simulink model "odrive_foc"  (R2024b)
settings: Solver=FixedStepDiscrete  StartTime=0  StopTime=4  FixedStep=5e-05  RelTol=1e-3
model workspace (MAT data in the model file):
  demo_load_nm = 0.0014
  demo_mode = 2
  demo_target = 2
  motor.R_ohm = 8
  motor.L_h = 0.00425
  motor.pole_pairs = 7
  motor.flux_wb = 0.003
  motor.inertia_kgm2 = 3e-05
  motor.damping_nms = 0.0003
undefined symbols (not defined in the file or in its folder): DiscIntNeverNeededParam
libraries: simulink x9
Description:
  | ODrive 3.6 three-loop bench. Export the FOC Motion Controller subsystem to the STM32.
settings Model: Creator=ODrive 3.6 Simulink FOC contributors  LastModifiedBy=ODrive 3.6 Simulink FOC contributors
settings DebuggingCC: AlgebraicLoopMsg=error

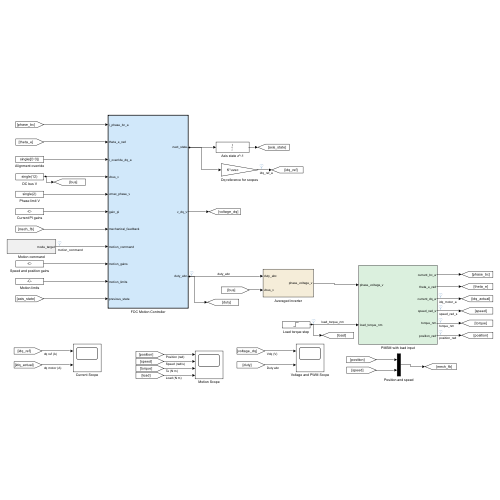
[thumbnail: Simulink's stored preview of the top-level diagram]
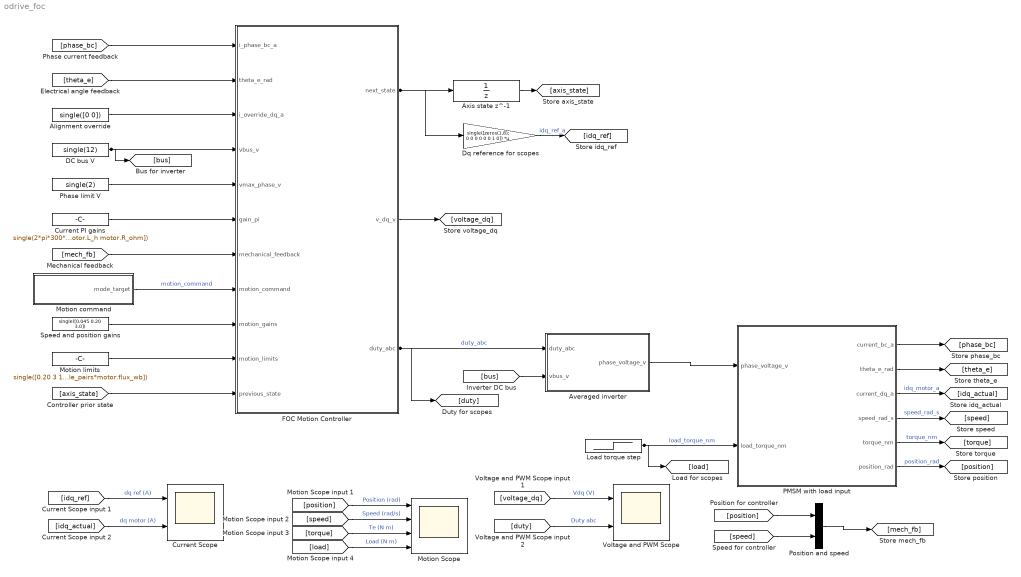
== system odrive_foc ==
  Alignment override : Constant  Value=single([0 0])
  Averaged inverter : Subsystem
  Axis state z^-1 : UnitDelay  InitialCondition=single(zeros(1,8))  SampleTime=5e-05
  Current PI gains : Constant  Value=single(2*pi*300*[motor.L_h motor.R_ohm motor.L_h motor.R_ohm])
  Current Scope : Scope  NumInputPorts=2
  DC bus V : Constant  Value=single(12)
  Dq reference for scopes : Gain  Gain=single([zeros(1,8); 0 0 0 0 0 0 1 0])  Multiplication=Matrix(K*u) (u vector)
  FOC Motion Controller : Subsystem  Description=Position P and speed PI at 1 kHz, current FOC and PWM at 20 kHz.  TreatAsAtomicUnit=on
  Load torque step : Step  Time=0.65  Before=single(0)  After=single(demo_load_nm)  OutDataTypeStr=single  SampleTime=5e-05
  Motion Scope : Scope  NumInputPorts=4
  Motion command : Subsystem
  Motion limits : Constant  Value=single([0.20 3 12 2 1.5*motor.pole_pairs*motor.flux_wb])
  PMSM with load input : Subsystem
  Phase limit V : Constant  Value=single(2)
  Position and speed : Mux  Inputs=2
  Speed and position gains : Constant  Value=single([0.045 0.20 3.0])
  Voltage and PWM Scope : Scope  NumInputPorts=2
  wires:
  [phase_bc] -> FOC Motion Controller/1(i_phase_bc_a)
  [theta_e] -> FOC Motion Controller/2(theta_e_rad)
  Alignment override/1 -> FOC Motion Controller/3(i_override_dq_a)
  DC bus V/1 -> FOC Motion Controller/4(vbus_v), [bus]
  Phase limit V/1 -> FOC Motion Controller/5(vmax_phase_v)
  Current PI gains/1 -> FOC Motion Controller/6(gain_pi)
  [mech_fb] -> FOC Motion Controller/7(mechanical_feedback)
  Motion command/1(mode_target) -> FOC Motion Controller/8(motion_command)  "motion_command"
  Speed and position gains/1 -> FOC Motion Controller/9(motion_gains)
  Motion limits/1 -> FOC Motion Controller/10(motion_limits)
  [axis_state] -> FOC Motion Controller/11(previous_state)
  FOC Motion Controller/1(next_state) -> Axis state z^-1/1, Dq reference for scopes/1
  Axis state z^-1/1 -> [axis_state]
  Dq reference for scopes/1 -> [idq_ref]  "idq_ref_a"
  FOC Motion Controller/2(v_dq_v) -> [voltage_dq]
  [bus] -> Averaged inverter/2(vbus_v)
  FOC Motion Controller/3(duty_abc) -> Averaged inverter/1(duty_abc), [duty]  "duty_abc"
  Averaged inverter/1(phase_voltage_v) -> PMSM with load input/1(phase_voltage_v)
  Load torque step/1 -> PMSM with load input/2(load_torque_nm), [load]  "load_torque_nm"
  PMSM with load input/1(current_bc_a) -> [phase_bc]
  PMSM with load input/2(theta_e_rad) -> [theta_e]
  PMSM with load input/3(current_dq_a) -> [idq_actual]  "idq_motor_a"
  PMSM with load input/4(speed_rad_s) -> [speed]  "speed_rad_s"
  PMSM with load input/5(torque_nm) -> [torque]  "torque_nm"
  PMSM with load input/6(position_rad) -> [position]  "position_rad"
  [position] -> Position and speed/1
  [speed] -> Position and speed/2
  Position and speed/1 -> [mech_fb]
  [idq_ref] -> Current Scope/1  "dq ref (A)"
  [idq_actual] -> Current Scope/2  "dq motor (A)"
  [position] -> Motion Scope/1  "Position (rad)"
  [speed] -> Motion Scope/2  "Speed (rad/s)"
  [torque] -> Motion Scope/3  "Te (N m)"
  [load] -> Motion Scope/4  "Load (N m)"
  [voltage_dq] -> Voltage and PWM Scope/1  "Vdq (V)"
  [duty] -> Voltage and PWM Scope/2  "Duty abc"

== system odrive_foc/Averaged inverter ==
  duty_abc : Inport
  vbus_v : Inport  Port=2
  Duty times DC bus : Product  Inputs=**
  Remove common mode : Gain  Gain=single(eye(3) - ones(3)/3)  Multiplication=Matrix(K*u) (u vector)
  phase_voltage_v : Outport
  wires:
  duty_abc/1 -> Remove common mode/1
  Remove common mode/1 -> Duty times DC bus/1
  vbus_v/1 -> Duty times DC bus/2
  Duty times DC bus/1 -> phase_voltage_v/1

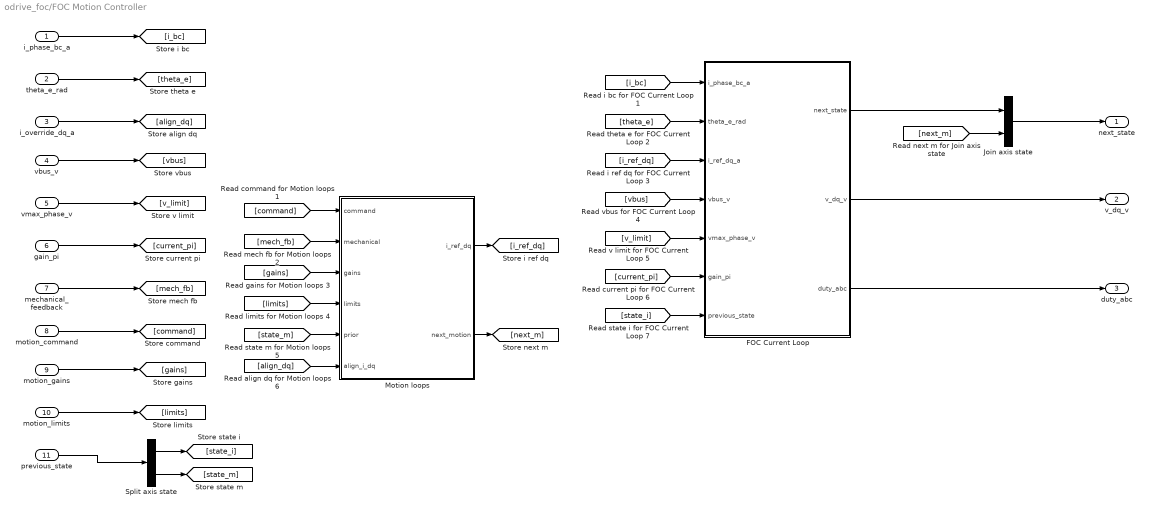
== system odrive_foc/FOC Motion Controller ==
  i_phase_bc_a : Inport  OutDataTypeStr=single  PortDimensions=2  SampleTime=5e-05  Interpolate=off
  theta_e_rad : Inport  Port=2  OutDataTypeStr=single  PortDimensions=1  SampleTime=5e-05  Interpolate=off
  i_override_dq_a : Inport  Port=3  OutDataTypeStr=single  PortDimensions=2  SampleTime=5e-05  Interpolate=off
  vbus_v : Inport  Port=4  OutDataTypeStr=single  PortDimensions=1  SampleTime=5e-05  Interpolate=off
  vmax_phase_v : Inport  Port=5  OutDataTypeStr=single  PortDimensions=1  SampleTime=5e-05  Interpolate=off
  gain_pi : Inport  Port=6  OutDataTypeStr=single  PortDimensions=4  SampleTime=5e-05  Interpolate=off
  mechanical_feedback : Inport  Port=7  OutDataTypeStr=single  PortDimensions=2  SampleTime=5e-05  Interpolate=off
  motion_command : Inport  Port=8  OutDataTypeStr=single  PortDimensions=2  SampleTime=5e-05  Interpolate=off
  motion_gains : Inport  Port=9  OutDataTypeStr=single  PortDimensions=3  SampleTime=5e-05  Interpolate=off
  motion_limits : Inport  Port=10  OutDataTypeStr=single  PortDimensions=5  SampleTime=5e-05  Interpolate=off
  previous_state : Inport  Port=11  OutDataTypeStr=single  PortDimensions=8  SampleTime=5e-05  Interpolate=off
  FOC Current Loop : Subsystem
  Join axis state : Mux  Inputs=2
  Motion loops : Subsystem
  Split axis state : Demux  Outputs=[4 4]
  next_state : Outport  OutDataTypeStr=single  PortDimensions=8
  v_dq_v : Outport  Port=2  OutDataTypeStr=single  PortDimensions=2
  duty_abc : Outport  Port=3  OutDataTypeStr=single  PortDimensions=3
  wires:
  i_phase_bc_a/1 -> [i_bc]
  theta_e_rad/1 -> [theta_e]
  i_override_dq_a/1 -> [align_dq]
  vbus_v/1 -> [vbus]
  vmax_phase_v/1 -> [v_limit]
  gain_pi/1 -> [current_pi]
  mechanical_feedback/1 -> [mech_fb]
  motion_command/1 -> [command]
  motion_gains/1 -> [gains]
  motion_limits/1 -> [limits]
  previous_state/1 -> Split axis state/1
  Split axis state/1 -> [state_i]
  Split axis state/2 -> [state_m]
  [command] -> Motion loops/1(command)
  [mech_fb] -> Motion loops/2(mechanical)
  [gains] -> Motion loops/3(gains)
  [limits] -> Motion loops/4(limits)
  [state_m] -> Motion loops/5(prior)
  [align_dq] -> Motion loops/6(align_i_dq)
  Motion loops/2(next_motion) -> [next_m]
  Motion loops/1(i_ref_dq) -> [i_ref_dq]
  [i_bc] -> FOC Current Loop/1(i_phase_bc_a)
  [theta_e] -> FOC Current Loop/2(theta_e_rad)
  [i_ref_dq] -> FOC Current Loop/3(i_ref_dq_a)
  [vbus] -> FOC Current Loop/4(vbus_v)
  [v_limit] -> FOC Current Loop/5(vmax_phase_v)
  [current_pi] -> FOC Current Loop/6(gain_pi)
  [state_i] -> FOC Current Loop/7(previous_state)
  FOC Current Loop/1(next_state) -> Join axis state/1
  [next_m] -> Join axis state/2
  Join axis state/1 -> next_state/1
  FOC Current Loop/2(v_dq_v) -> v_dq_v/1
  FOC Current Loop/3(duty_abc) -> duty_abc/1

== system odrive_foc/Motion command ==
  Mode 1 torque 2 speed 3 position : Constant  Value=single(demo_mode)
  Mode and target : Mux  Inputs=2
  Target step : Step  Time=0.04  Before=single(0)  After=single(demo_target)  OutDataTypeStr=single  SampleTime=5e-05
  mode_target : Outport
  wires:
  Mode 1 torque 2 speed 3 position/1 -> Mode and target/1
  Target step/1 -> Mode and target/2
  Mode and target/1 -> mode_target/1

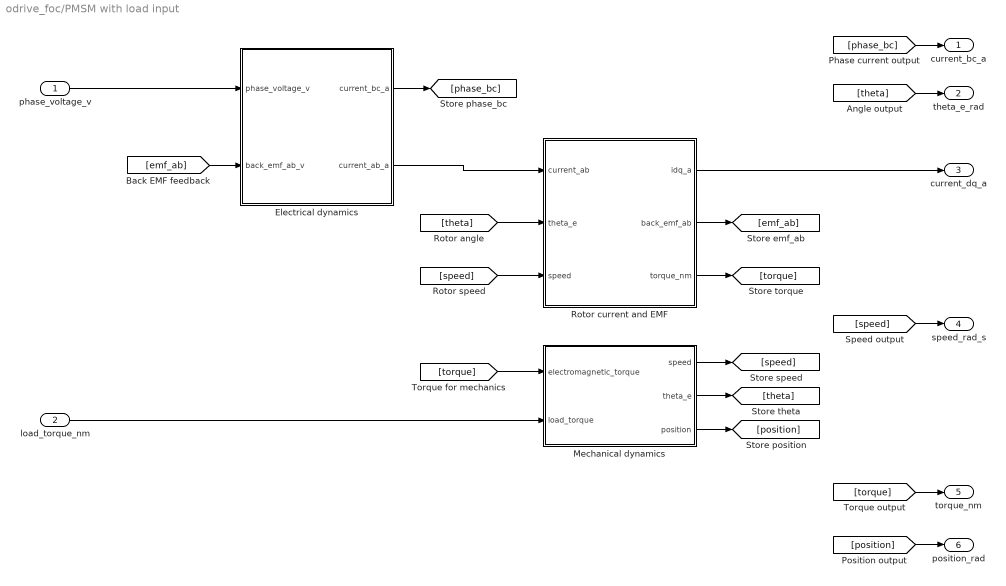
== system odrive_foc/PMSM with load input ==
  phase_voltage_v : Inport
  load_torque_nm : Inport  Port=2
  Electrical dynamics : Subsystem
  Mechanical dynamics : Subsystem
  Rotor current and EMF : Subsystem
  current_bc_a : Outport
  theta_e_rad : Outport  Port=2
  current_dq_a : Outport  Port=3
  speed_rad_s : Outport  Port=4
  torque_nm : Outport  Port=5
  position_rad : Outport  Port=6
  wires:
  phase_voltage_v/1 -> Electrical dynamics/1(phase_voltage_v)
  Electrical dynamics/2(current_ab_a) -> Rotor current and EMF/1(current_ab)
  load_torque_nm/1 -> Mechanical dynamics/2(load_torque)
  Rotor current and EMF/1(idq_a) -> current_dq_a/1
  Electrical dynamics/1(current_bc_a) -> [phase_bc]
  Rotor current and EMF/2(back_emf_ab) -> [emf_ab]
  Rotor current and EMF/3(torque_nm) -> [torque]
  Mechanical dynamics/1(speed) -> [speed]
  Mechanical dynamics/2(theta_e) -> [theta]
  Mechanical dynamics/3(position) -> [position]
  [emf_ab] -> Electrical dynamics/2(back_emf_ab_v)
  [theta] -> Rotor current and EMF/2(theta_e)
  [speed] -> Rotor current and EMF/3(speed)
  [torque] -> Mechanical dynamics/1(electromagnetic_torque)
  [phase_bc] -> current_bc_a/1
  [theta] -> theta_e_rad/1
  [speed] -> speed_rad_s/1
  [torque] -> torque_nm/1
  [position] -> position_rad/1

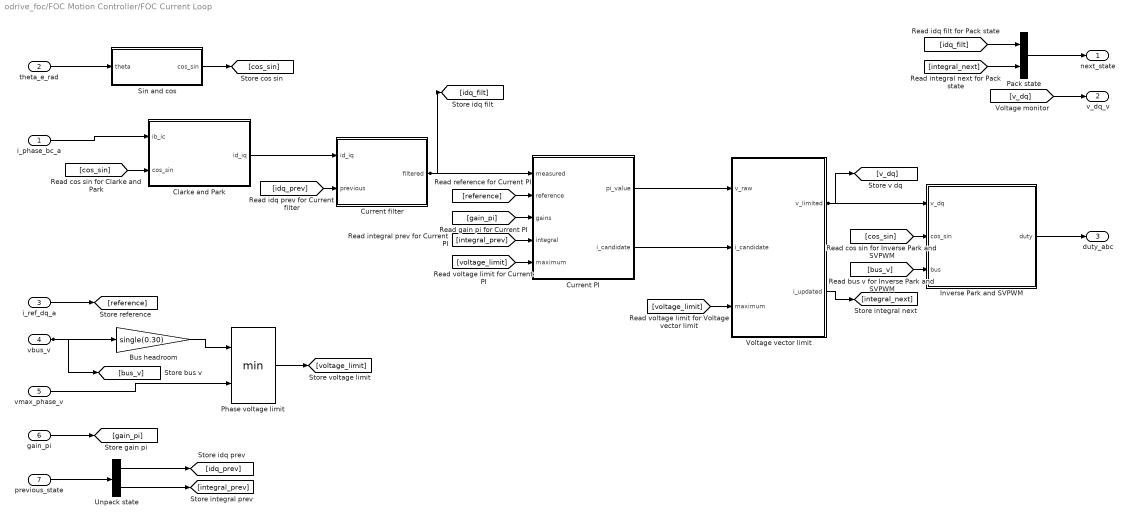
== system odrive_foc/FOC Motion Controller/FOC Current Loop ==
  i_phase_bc_a : Inport  OutDataTypeStr=single  PortDimensions=2  SampleTime=5e-05  Interpolate=off
  theta_e_rad : Inport  Port=2  OutDataTypeStr=single  PortDimensions=1  SampleTime=5e-05  Interpolate=off
  i_ref_dq_a : Inport  Port=3  OutDataTypeStr=single  PortDimensions=2  SampleTime=5e-05  Interpolate=off
  vbus_v : Inport  Port=4  OutDataTypeStr=single  PortDimensions=1  SampleTime=5e-05  Interpolate=off
  vmax_phase_v : Inport  Port=5  OutDataTypeStr=single  PortDimensions=1  SampleTime=5e-05  Interpolate=off
  gain_pi : Inport  Port=6  OutDataTypeStr=single  PortDimensions=4  SampleTime=5e-05  Interpolate=off
  previous_state : Inport  Port=7  OutDataTypeStr=single  PortDimensions=4  SampleTime=5e-05  Interpolate=off
  Bus headroom : Gain  Gain=single(0.30)
  Clarke and Park : Subsystem
  Current PI : Subsystem
  Current filter : Subsystem
  Inverse Park and SVPWM : Subsystem
  Pack state : Mux  Inputs=2
  Phase voltage limit : MinMax  Inputs=2
  Sin and cos : Subsystem
  Unpack state : Demux  Outputs=[2 2]
  Voltage vector limit : Subsystem
  next_state : Outport  OutDataTypeStr=single  PortDimensions=4
  v_dq_v : Outport  Port=2  OutDataTypeStr=single  PortDimensions=2
  duty_abc : Outport  Port=3  OutDataTypeStr=single  PortDimensions=3
  wires:
  Sin and cos/1(cos_sin) -> [cos_sin]
  theta_e_rad/1 -> Sin and cos/1(theta)
  [cos_sin] -> Clarke and Park/2(cos_sin)
  i_phase_bc_a/1 -> Clarke and Park/1(ib_ic)
  [idq_prev] -> Current filter/2(previous)
  Clarke and Park/1(id_iq) -> Current filter/1(id_iq)
  Current filter/1(filtered) -> [idq_filt], Current PI/1(measured)
  [reference] -> Current PI/2(reference)
  [gain_pi] -> Current PI/3(gains)
  [integral_prev] -> Current PI/4(integral)
  [voltage_limit] -> Current PI/5(maximum)
  Current PI/1(pi_value) -> Voltage vector limit/1(v_raw)
  Current PI/2(i_candidate) -> Voltage vector limit/2(i_candidate)
  [voltage_limit] -> Voltage vector limit/3(maximum)
  Voltage vector limit/1(v_limited) -> [v_dq], Inverse Park and SVPWM/1(v_dq)
  Voltage vector limit/2(i_updated) -> [integral_next]
  [cos_sin] -> Inverse Park and SVPWM/2(cos_sin)
  [bus_v] -> Inverse Park and SVPWM/3(bus)
  Inverse Park and SVPWM/1(duty) -> duty_abc/1
  [v_dq] -> v_dq_v/1
  [idq_filt] -> Pack state/1
  [integral_next] -> Pack state/2
  Pack state/1 -> next_state/1
  i_ref_dq_a/1 -> [reference]
  gain_pi/1 -> [gain_pi]
  previous_state/1 -> Unpack state/1
  Unpack state/1 -> [idq_prev]
  Unpack state/2 -> [integral_prev]
  vbus_v/1 -> Bus headroom/1, [bus_v]
  Bus headroom/1 -> Phase voltage limit/1
  vmax_phase_v/1 -> Phase voltage limit/2
  Phase voltage limit/1 -> [voltage_limit]

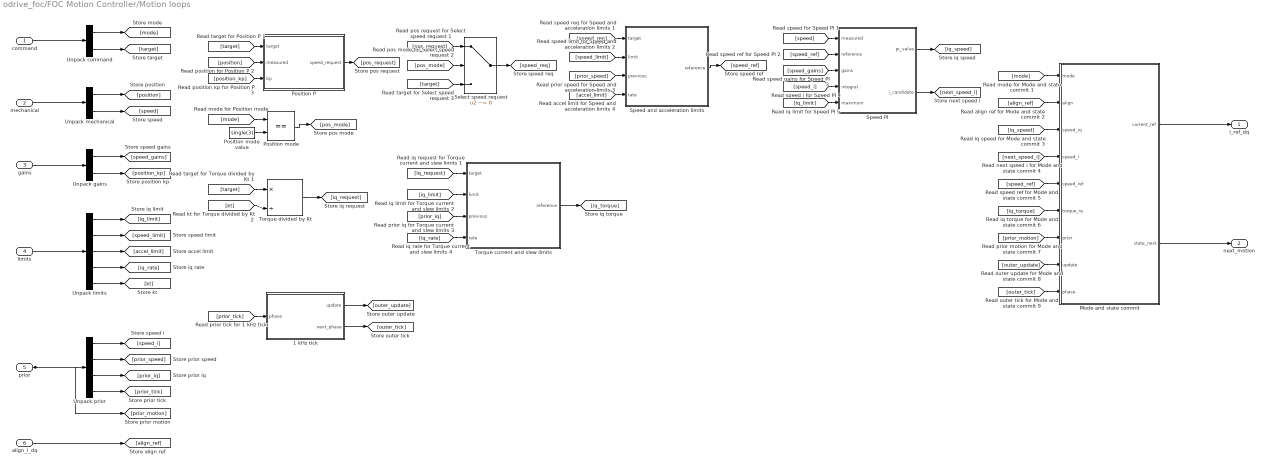
== system odrive_foc/FOC Motion Controller/Motion loops ==
  command : Inport
  mechanical : Inport  Port=2
  gains : Inport  Port=3
  limits : Inport  Port=4
  prior : Inport  Port=5
  align_i_dq : Inport  Port=6
  1 kHz tick : Subsystem
  Mode and state commit : Subsystem
  Position P : Subsystem
  Position mode : RelationalOperator  Operator===
  Position mode value : Constant  Value=single(3)
  Select speed request : Switch  Criteria=u2 ~= 0
  Speed PI : Subsystem
  Speed and acceleration limits : Subsystem
  Torque current and slew limits : Subsystem
  Torque divided by Kt : Product  Inputs=*/
  Unpack command : Demux  Outputs=[1 1]
  Unpack gains : Demux  Outputs=[2 1]
  Unpack limits : Demux  Outputs=[1 1 1 1 1]
  Unpack mechanical : Demux  Outputs=[1 1]
  Unpack prior : Demux  Outputs=[1 1 1 1]
  i_ref_dq : Outport
  next_motion : Outport  Port=2
  wires:
  command/1 -> Unpack command/1
  Unpack command/1 -> [mode]
  Unpack command/2 -> [target]
  mechanical/1 -> Unpack mechanical/1
  Unpack mechanical/1 -> [position]
  Unpack mechanical/2 -> [speed]
  gains/1 -> Unpack gains/1
  Unpack gains/1 -> [speed_gains]
  Unpack gains/2 -> [position_kp]
  limits/1 -> Unpack limits/1
  Unpack limits/1 -> [iq_limit]
  Unpack limits/2 -> [speed_limit]
  Unpack limits/3 -> [accel_limit]
  Unpack limits/4 -> [iq_rate]
  Unpack limits/5 -> [kt]
  prior/1 -> Unpack prior/1, [prior_motion]
  Unpack prior/1 -> [speed_i]
  Unpack prior/2 -> [prior_speed]
  Unpack prior/3 -> [prior_iq]
  Unpack prior/4 -> [prior_tick]
  align_i_dq/1 -> [align_ref]
  [target] -> Position P/1(target)
  [position] -> Position P/2(measured)
  [position_kp] -> Position P/3(kp)
  Position P/1(speed_request) -> [pos_request]
  [mode] -> Position mode/1
  Position mode value/1 -> Position mode/2
  Position mode/1 -> [pos_mode]
  [pos_request] -> Select speed request/1
  [pos_mode] -> Select speed request/2
  [target] -> Select speed request/3
  Select speed request/1 -> [speed_req]
  [speed_req] -> Speed and acceleration limits/1(target)
  [speed_limit] -> Speed and acceleration limits/2(limit)
  [prior_speed] -> Speed and acceleration limits/3(previous)
  [accel_limit] -> Speed and acceleration limits/4(rate)
  Speed and acceleration limits/1(reference) -> [speed_ref]
  [speed] -> Speed PI/1(measured)
  [speed_ref] -> Speed PI/2(reference)
  [speed_gains] -> Speed PI/3(gains)
  [speed_i] -> Speed PI/4(integral)
  [iq_limit] -> Speed PI/5(maximum)
  Speed PI/1(pi_value) -> [iq_speed]
  Speed PI/2(i_candidate) -> [next_speed_i]
  [target] -> Torque divided by Kt/1
  [kt] -> Torque divided by Kt/2
  Torque divided by Kt/1 -> [iq_request]
  [iq_request] -> Torque current and slew limits/1(target)
  [iq_limit] -> Torque current and slew limits/2(limit)
  [prior_iq] -> Torque current and slew limits/3(previous)
  [iq_rate] -> Torque current and slew limits/4(rate)
  Torque current and slew limits/1(reference) -> [iq_torque]
  [prior_tick] -> 1 kHz tick/1(phase)
  1 kHz tick/1(update) -> [outer_update]
  1 kHz tick/2(next_phase) -> [outer_tick]
  [mode] -> Mode and state commit/1(mode)
  [align_ref] -> Mode and state commit/2(align)
  [iq_speed] -> Mode and state commit/3(speed_iq)
  [next_speed_i] -> Mode and state commit/4(speed_i)
  [speed_ref] -> Mode and state commit/5(speed_ref)
  [iq_torque] -> Mode and state commit/6(torque_iq)
  [prior_motion] -> Mode and state commit/7(prior)
  [outer_update] -> Mode and state commit/8(update)
  [outer_tick] -> Mode and state commit/9(phase)
  Mode and state commit/1(current_ref) -> i_ref_dq/1
  Mode and state commit/2(state_next) -> next_motion/1

== system odrive_foc/PMSM with load input/Electrical dynamics ==
  phase_voltage_v : Inport
  back_emf_ab_v : Inport  Port=2
  Clarke voltage : Gain  Gain=single([2/3 -1/3 -1/3; 0 1/sqrt(3) -1/sqrt(3)])  Multiplication=Matrix(K*u) (u vector)
  Inverse Clarke B C : Gain  Gain=single([-0.5 sqrt(3)/2; -0.5 -sqrt(3)/2])  Multiplication=Matrix(K*u) (u vector)
  Winding current : DiscreteIntegrator  gainval=1/motor.L_h  InitialCondition=single(0)  SampleTime=5e-05  ICPrevOutput=DiscIntNeverNeededParam  ICPrevScaledInput=DiscIntNeverNeededParam
  Winding resistance : Gain  Gain=single(motor.R_ohm)
  Winding voltage : Sum  Inputs=+--
  current_bc_a : Outport
  current_ab_a : Outport  Port=2
  wires:
  Winding current/1 -> [current_ab], current_ab_a/1, Inverse Clarke B C/1
  [current_ab] -> Winding resistance/1
  phase_voltage_v/1 -> Clarke voltage/1
  Clarke voltage/1 -> Winding voltage/1
  Winding resistance/1 -> Winding voltage/2
  back_emf_ab_v/1 -> Winding voltage/3
  Winding voltage/1 -> Winding current/1
  Inverse Clarke B C/1 -> current_bc_a/1

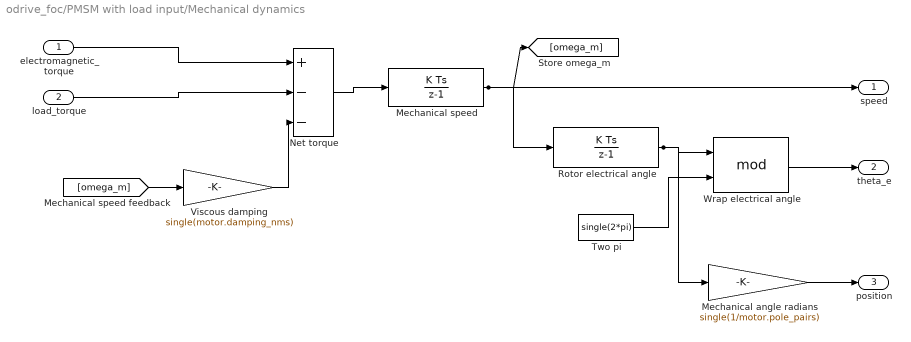
== system odrive_foc/PMSM with load input/Mechanical dynamics ==
  electromagnetic_torque : Inport
  load_torque : Inport  Port=2
  Mechanical angle radians : Gain  Gain=single(1/motor.pole_pairs)
  Mechanical speed : DiscreteIntegrator  gainval=1/motor.inertia_kgm2  InitialCondition=single(0)  SampleTime=5e-05  ICPrevOutput=DiscIntNeverNeededParam  ICPrevScaledInput=DiscIntNeverNeededParam
  Net torque : Sum  Inputs=+--
  Rotor electrical angle : DiscreteIntegrator  gainval=motor.pole_pairs  InitialCondition=single(0)  SampleTime=5e-05  ICPrevOutput=DiscIntNeverNeededParam  ICPrevScaledInput=DiscIntNeverNeededParam
  Two pi : Constant  Value=single(2*pi)
  Viscous damping : Gain  Gain=single(motor.damping_nms)
  Wrap electrical angle : Math  Operator=mod
  speed : Outport
  theta_e : Outport  Port=2
  position : Outport  Port=3
  wires:
  Mechanical speed/1 -> [omega_m], speed/1, Rotor electrical angle/1
  [omega_m] -> Viscous damping/1
  electromagnetic_torque/1 -> Net torque/1
  load_torque/1 -> Net torque/2
  Viscous damping/1 -> Net torque/3
  Net torque/1 -> Mechanical speed/1
  Rotor electrical angle/1 -> Wrap electrical angle/1, Mechanical angle radians/1
  Two pi/1 -> Wrap electrical angle/2
  Mechanical angle radians/1 -> position/1
  Wrap electrical angle/1 -> theta_e/1

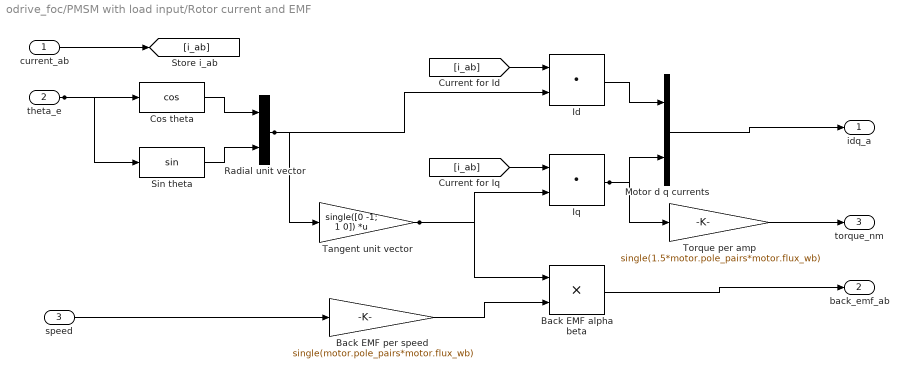
== system odrive_foc/PMSM with load input/Rotor current and EMF ==
  current_ab : Inport
  theta_e : Inport  Port=2
  speed : Inport  Port=3
  Back EMF alpha beta : Product  Inputs=**
  Back EMF per speed : Gain  Gain=single(motor.pole_pairs*motor.flux_wb)
  Cos theta : Trigonometry  Operator=cos
  Id : DotProduct  OutDataTypeStr=Inherit: Inherit via internal rule
  Iq : DotProduct  OutDataTypeStr=Inherit: Inherit via internal rule
  Motor d q currents : Mux  Inputs=2
  Radial unit vector : Mux  Inputs=2
  Sin theta : Trigonometry
  Tangent unit vector : Gain  Gain=single([0 -1; 1 0])  Multiplication=Matrix(K*u) (u vector)
  Torque per amp : Gain  Gain=single(1.5*motor.pole_pairs*motor.flux_wb)
  idq_a : Outport
  back_emf_ab : Outport  Port=2
  torque_nm : Outport  Port=3
  wires:
  current_ab/1 -> [i_ab]
  [i_ab] -> Id/1
  [i_ab] -> Iq/1
  theta_e/1 -> Cos theta/1, Sin theta/1
  Cos theta/1 -> Radial unit vector/1
  Sin theta/1 -> Radial unit vector/2
  Radial unit vector/1 -> Id/2, Tangent unit vector/1
  Tangent unit vector/1 -> Iq/2, Back EMF alpha beta/1
  Id/1 -> Motor d q currents/1
  Iq/1 -> Motor d q currents/2, Torque per amp/1
  Motor d q currents/1 -> idq_a/1
  Torque per amp/1 -> torque_nm/1
  speed/1 -> Back EMF per speed/1
  Back EMF per speed/1 -> Back EMF alpha beta/2
  Back EMF alpha beta/1 -> back_emf_ab/1

== system odrive_foc/FOC Motion Controller/FOC Current Loop/Clarke and Park ==
  ib_ic : Inport
  cos_sin : Inport  Port=2
  Clarke B C to alpha beta : Gain  Gain=single([-1 -1; 0.57735026919 -0.57735026919])  Multiplication=Matrix(K*u) (u vector)
  Park rotation : Subsystem
  id_iq : Outport
  wires:
  ib_ic/1 -> Clarke B C to alpha beta/1
  Clarke B C to alpha beta/1 -> Park rotation/1(stationary)
  cos_sin/1 -> Park rotation/2(cos_sin)
  Park rotation/1(rotating) -> id_iq/1

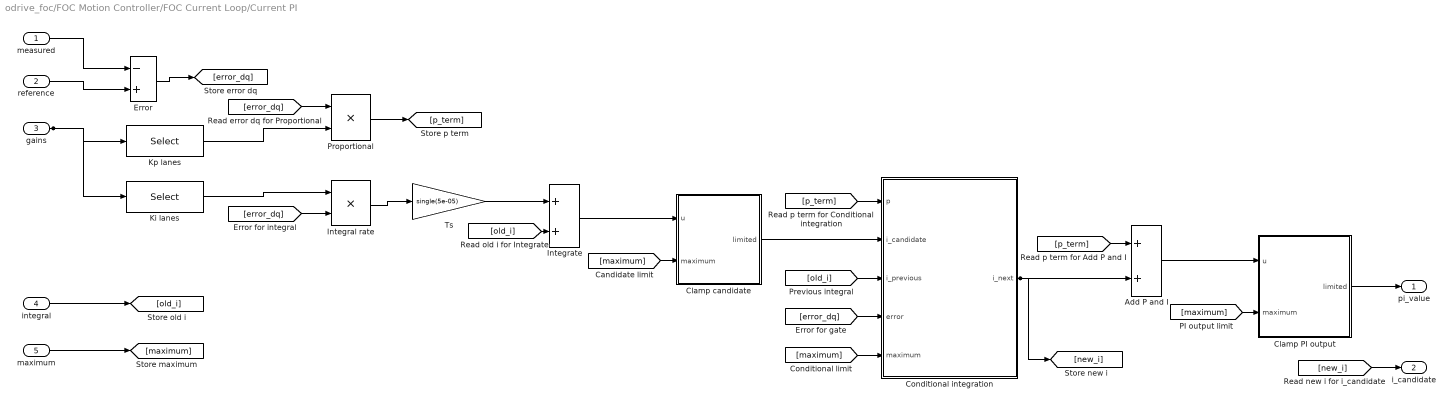
== system odrive_foc/FOC Motion Controller/FOC Current Loop/Current PI ==
  measured : Inport
  reference : Inport  Port=2
  gains : Inport  Port=3
  integral : Inport  Port=4
  maximum : Inport  Port=5
  Add P and I : Sum
  Clamp PI output : Subsystem
  Clamp candidate : Subsystem
  Conditional integration : Subsystem
  Error : Sum  Inputs=-+
  Integral rate : Product  Inputs=**
  Integrate : Sum
  Ki lanes : Selector  InputPortWidth=4  IndexOptions=Index vector (dialog)  Indices=[2 4]  OutputSizes=1
  Kp lanes : Selector  InputPortWidth=4  IndexOptions=Index vector (dialog)  Indices=[1 3]  OutputSizes=1
  Proportional : Product  Inputs=**
  Ts : Gain  Gain=single(5e-05)
  pi_value : Outport
  i_candidate : Outport  Port=2
  wires:
  Error/1 -> [error_dq]
  integral/1 -> [old_i]
  maximum/1 -> [maximum]
  measured/1 -> Error/1
  reference/1 -> Error/2
  gains/1 -> Kp lanes/1, Ki lanes/1
  Proportional/1 -> [p_term]
  [error_dq] -> Proportional/1
  [error_dq] -> Integral rate/2
  Kp lanes/1 -> Proportional/2
  Ki lanes/1 -> Integral rate/1
  [old_i] -> Integrate/2
  Integral rate/1 -> Ts/1
  Ts/1 -> Integrate/1
  Integrate/1 -> Clamp candidate/1(u)
  [maximum] -> Clamp candidate/2(maximum)
  Clamp candidate/1(limited) -> Conditional integration/2(i_candidate)
  [p_term] -> Conditional integration/1(p)
  [old_i] -> Conditional integration/3(i_previous)
  [error_dq] -> Conditional integration/4(error)
  [maximum] -> Conditional integration/5(maximum)
  [p_term] -> Add P and I/1
  [maximum] -> Clamp PI output/2(maximum)
  Conditional integration/1(i_next) -> [new_i], Add P and I/2
  [new_i] -> i_candidate/1
  Add P and I/1 -> Clamp PI output/1(u)
  Clamp PI output/1(limited) -> pi_value/1

== system odrive_foc/FOC Motion Controller/FOC Current Loop/Current filter ==
  id_iq : Inport
  previous : Inport  Port=2
  Current delta : Sum  Inputs=+-
  Filter coefficient : Gain  Gain=single(0.15)
  Update filter : Sum
  filtered : Outport
  wires:
  previous/1 -> [prior]
  [prior] -> Current delta/2
  [prior] -> Update filter/2
  id_iq/1 -> Current delta/1
  Current delta/1 -> Filter coefficient/1
  Filter coefficient/1 -> Update filter/1
  Update filter/1 -> filtered/1

== system odrive_foc/FOC Motion Controller/FOC Current Loop/Inverse Park and SVPWM ==
  v_dq : Inport
  cos_sin : Inport  Port=2
  bus : Inport  Port=3
  Common mode : Subsystem
  Inverse Park rotation : Subsystem
  Midpoint : Bias  Bias=single(0.5)
  Minimum bus : Constant  Value=single(1)
  Normalize by bus : Product  Inputs=*/
  PWM duty bounds : Saturate  UpperLimit=single(0.80)  LowerLimit=single(0.10)
  Phase voltages : Gain  Gain=single([1 0; -0.5 0.86602540378; -0.5 -0.86602540378])  Multiplication=Matrix(K*u) (u vector)
  Remove common mode : Sum  Inputs=+-
  Safe bus : MinMax  Function=max  Inputs=2
  duty : Outport
  wires:
  v_dq/1 -> Inverse Park rotation/1(rotating)
  cos_sin/1 -> Inverse Park rotation/2(cos_sin)
  Inverse Park rotation/1(stationary) -> Phase voltages/1
  Phase voltages/1 -> Common mode/1(phase_volts), Remove common mode/1
  Common mode/1(common_voltage) -> Remove common mode/2
  Minimum bus/1 -> Safe bus/1
  bus/1 -> Safe bus/2
  Remove common mode/1 -> Normalize by bus/1
  Safe bus/1 -> Normalize by bus/2
  Normalize by bus/1 -> Midpoint/1
  Midpoint/1 -> PWM duty bounds/1
  PWM duty bounds/1 -> duty/1

== system odrive_foc/FOC Motion Controller/FOC Current Loop/Sin and cos ==
  theta : Inport
  Cos sin : Mux  Inputs=2
  Cosine : Trigonometry  Operator=cos
  Sine : Trigonometry
  cos_sin : Outport
  wires:
  theta/1 -> Cosine/1, Sine/1
  Cosine/1 -> Cos sin/1
  Sine/1 -> Cos sin/2
  Cos sin/1 -> cos_sin/1

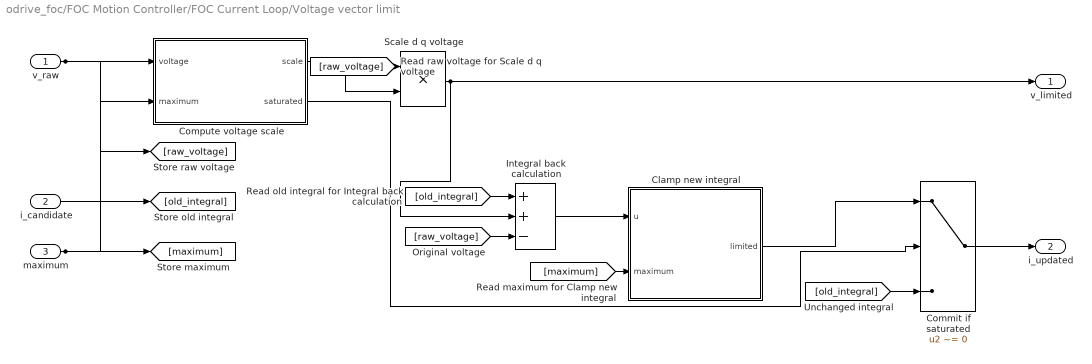
== system odrive_foc/FOC Motion Controller/FOC Current Loop/Voltage vector limit ==
  v_raw : Inport
  i_candidate : Inport  Port=2
  maximum : Inport  Port=3
  Clamp new integral : Subsystem
  Commit if saturated : Switch  Criteria=u2 ~= 0
  Compute voltage scale : Subsystem
  Integral back calculation : Sum  Inputs=++-
  Scale d q voltage : Product  Inputs=**
  v_limited : Outport
  i_updated : Outport  Port=2
  wires:
  v_raw/1 -> [raw_voltage], Compute voltage scale/1(voltage)
  i_candidate/1 -> [old_integral]
  maximum/1 -> [maximum], Compute voltage scale/2(maximum)
  [raw_voltage] -> Scale d q voltage/1
  [old_integral] -> Integral back calculation/1
  [raw_voltage] -> Integral back calculation/3
  [maximum] -> Clamp new integral/2(maximum)
  [old_integral] -> Commit if saturated/3
  Compute voltage scale/1(scale) -> Scale d q voltage/2
  Scale d q voltage/1 -> v_limited/1, Integral back calculation/2
  Integral back calculation/1 -> Clamp new integral/1(u)
  Clamp new integral/1(limited) -> Commit if saturated/1
  Compute voltage scale/2(saturated) -> Commit if saturated/2
  Commit if saturated/1 -> i_updated/1

== system odrive_foc/FOC Motion Controller/Motion loops/1 kHz tick ==
  phase : Inport
  Base tick : Constant  Value=single(1)
  First tick : Constant  Value=single(0)
  Increment tick : Sum
  Outer update : RelationalOperator
  Ticks per update : Constant  Value=single(20)
  Wrap phase : Switch  Criteria=u2 ~= 0
  update : Outport
  next_phase : Outport  Port=2
  wires:
  Increment tick/1 -> [increment], Outer update/1
  Outer update/1 -> [update_signal], update/1
  [update_signal] -> Wrap phase/2
  [increment] -> Wrap phase/3
  phase/1 -> Increment tick/1
  Base tick/1 -> Increment tick/2
  Ticks per update/1 -> Outer update/2
  First tick/1 -> Wrap phase/1
  Wrap phase/1 -> next_phase/1

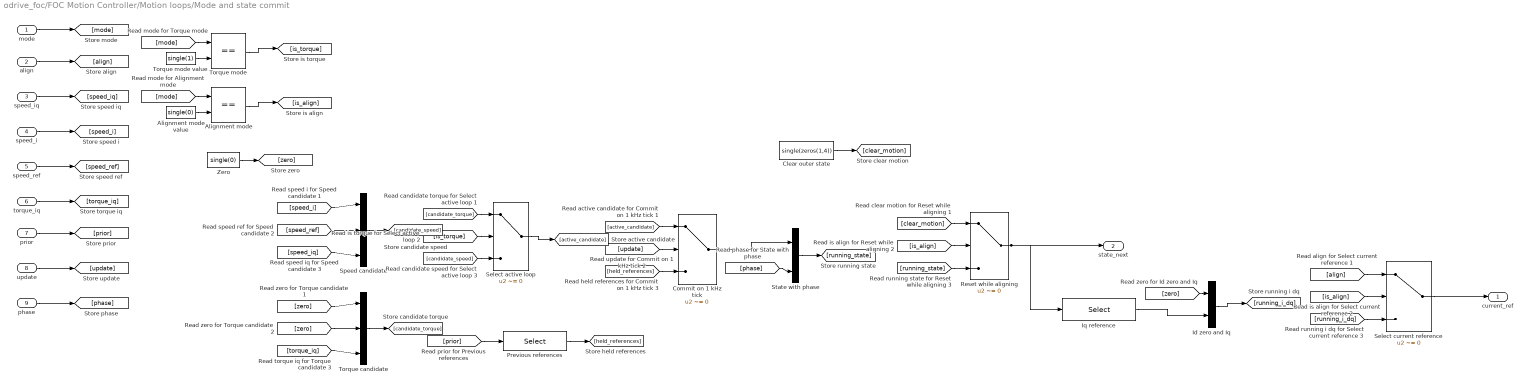
== system odrive_foc/FOC Motion Controller/Motion loops/Mode and state commit ==
  mode : Inport
  align : Inport  Port=2
  speed_iq : Inport  Port=3
  speed_i : Inport  Port=4
  speed_ref : Inport  Port=5
  torque_iq : Inport  Port=6
  prior : Inport  Port=7
  update : Inport  Port=8
  phase : Inport  Port=9
  Alignment mode : RelationalOperator  Operator===
  Alignment mode value : Constant  Value=single(0)
  Clear outer state : Constant  Value=single(zeros(1,4))
  Commit on 1 kHz tick : Switch  Criteria=u2 ~= 0
  Id zero and Iq : Mux  Inputs=2
  Iq reference : Selector  InputPortWidth=4  IndexOptions=Index vector (dialog)  Indices=3  OutputSizes=1
  Previous references : Selector  InputPortWidth=4  IndexOptions=Index vector (dialog)  Indices=[1 2 3]  OutputSizes=1
  Reset while aligning : Switch  Criteria=u2 ~= 0
  Select active loop : Switch  Criteria=u2 ~= 0
  Select current reference : Switch  Criteria=u2 ~= 0
  Speed candidate : Mux  Inputs=3
  State with phase : Mux  Inputs=2
  Torque candidate : Mux  Inputs=3
  Torque mode : RelationalOperator  Operator===
  Torque mode value : Constant  Value=single(1)
  Zero : Constant  Value=single(0)
  current_ref : Outport
  state_next : Outport  Port=2
  wires:
  mode/1 -> [mode]
  align/1 -> [align]
  speed_iq/1 -> [speed_iq]
  speed_i/1 -> [speed_i]
  speed_ref/1 -> [speed_ref]
  torque_iq/1 -> [torque_iq]
  prior/1 -> [prior]
  update/1 -> [update]
  phase/1 -> [phase]
  Zero/1 -> [zero]
  [mode] -> Torque mode/1
  Torque mode value/1 -> Torque mode/2
  [mode] -> Alignment mode/1
  Alignment mode value/1 -> Alignment mode/2
  Torque mode/1 -> [is_torque]
  Alignment mode/1 -> [is_align]
  [speed_i] -> Speed candidate/1
  [speed_ref] -> Speed candidate/2
  [speed_iq] -> Speed candidate/3
  [zero] -> Torque candidate/1
  [zero] -> Torque candidate/2
  [torque_iq] -> Torque candidate/3
  Speed candidate/1 -> [candidate_speed]
  Torque candidate/1 -> [candidate_torque]
  [candidate_torque] -> Select active loop/1
  [is_torque] -> Select active loop/2
  [candidate_speed] -> Select active loop/3
  Select active loop/1 -> [active_candidate]
  [prior] -> Previous references/1
  Previous references/1 -> [held_references]
  [active_candidate] -> Commit on 1 kHz tick/1
  [update] -> Commit on 1 kHz tick/2
  [held_references] -> Commit on 1 kHz tick/3
  Commit on 1 kHz tick/1 -> State with phase/1
  [phase] -> State with phase/2
  State with phase/1 -> [running_state]
  Clear outer state/1 -> [clear_motion]
  [clear_motion] -> Reset while aligning/1
  [is_align] -> Reset while aligning/2
  [running_state] -> Reset while aligning/3
  Reset while aligning/1 -> state_next/1, Iq reference/1
  [zero] -> Id zero and Iq/1
  Iq reference/1 -> Id zero and Iq/2
  Id zero and Iq/1 -> [running_i_dq]
  [align] -> Select current reference/1
  [is_align] -> Select current reference/2
  [running_i_dq] -> Select current reference/3
  Select current reference/1 -> current_ref/1

== system odrive_foc/FOC Motion Controller/Motion loops/Position P ==
  target : Inport
  measured : Inport  Port=2
  kp : Inport  Port=3
  P gain : Product  Inputs=**
  Position error : Sum  Inputs=+-
  speed_request : Outport
  wires:
  target/1 -> Position error/1
  measured/1 -> Position error/2
  Position error/1 -> P gain/1
  kp/1 -> P gain/2
  P gain/1 -> speed_request/1

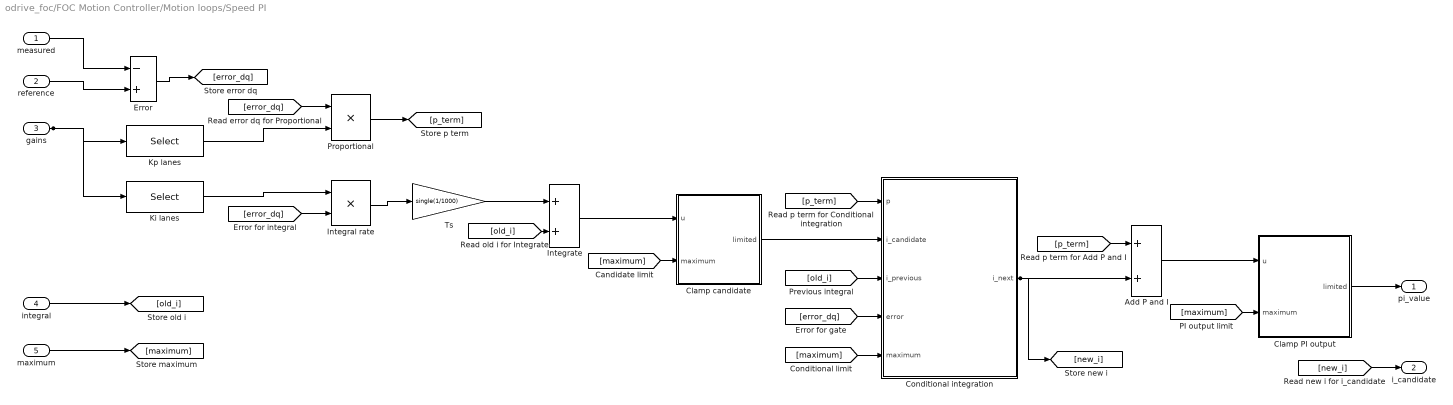
== system odrive_foc/FOC Motion Controller/Motion loops/Speed PI ==
  measured : Inport
  reference : Inport  Port=2
  gains : Inport  Port=3
  integral : Inport  Port=4
  maximum : Inport  Port=5
  Add P and I : Sum
  Clamp PI output : Subsystem
  Clamp candidate : Subsystem
  Conditional integration : Subsystem
  Error : Sum  Inputs=-+
  Integral rate : Product  Inputs=**
  Integrate : Sum
  Ki lanes : Selector  InputPortWidth=2  IndexOptions=Index vector (dialog)  Indices=2  OutputSizes=1
  Kp lanes : Selector  InputPortWidth=2  IndexOptions=Index vector (dialog)  Indices=1  OutputSizes=1
  Proportional : Product  Inputs=**
  Ts : Gain  Gain=single(1/1000)
  pi_value : Outport
  i_candidate : Outport  Port=2
  wires:
  Error/1 -> [error_dq]
  integral/1 -> [old_i]
  maximum/1 -> [maximum]
  measured/1 -> Error/1
  reference/1 -> Error/2
  gains/1 -> Kp lanes/1, Ki lanes/1
  Proportional/1 -> [p_term]
  [error_dq] -> Proportional/1
  [error_dq] -> Integral rate/2
  Kp lanes/1 -> Proportional/2
  Ki lanes/1 -> Integral rate/1
  [old_i] -> Integrate/2
  Integral rate/1 -> Ts/1
  Ts/1 -> Integrate/1
  Integrate/1 -> Clamp candidate/1(u)
  [maximum] -> Clamp candidate/2(maximum)
  Clamp candidate/1(limited) -> Conditional integration/2(i_candidate)
  [p_term] -> Conditional integration/1(p)
  [old_i] -> Conditional integration/3(i_previous)
  [error_dq] -> Conditional integration/4(error)
  [maximum] -> Conditional integration/5(maximum)
  [p_term] -> Add P and I/1
  [maximum] -> Clamp PI output/2(maximum)
  Conditional integration/1(i_next) -> [new_i], Add P and I/2
  [new_i] -> i_candidate/1
  Add P and I/1 -> Clamp PI output/1(u)
  Clamp PI output/1(limited) -> pi_value/1

== system odrive_foc/FOC Motion Controller/Motion loops/Speed and acceleration limits ==
  target : Inport
  limit : Inport  Port=2
  previous : Inport  Port=3
  rate : Inport  Port=4
  Apply step : Sum
  Limit rate : Subsystem
  Limit setpoint : Subsystem
  Step error : Sum  Inputs=+-
  Step time : Gain  Gain=single(1/1000)
  reference : Outport
  wires:
  previous/1 -> [previous_step]
  [previous_step] -> Step error/2
  [previous_step] -> Apply step/2
  target/1 -> Limit setpoint/1(u)
  limit/1 -> Limit setpoint/2(maximum)
  Limit setpoint/1(limited) -> Step error/1
  Step error/1 -> Limit rate/1(u)
  rate/1 -> Step time/1
  Step time/1 -> Limit rate/2(maximum)
  Limit rate/1(limited) -> Apply step/1
  Apply step/1 -> reference/1

== system odrive_foc/FOC Motion Controller/Motion loops/Torque current and slew limits ==
  target : Inport
  limit : Inport  Port=2
  previous : Inport  Port=3
  rate : Inport  Port=4
  Apply step : Sum
  Limit rate : Subsystem
  Limit setpoint : Subsystem
  Step error : Sum  Inputs=+-
  Step time : Gain  Gain=single(1/1000)
  reference : Outport
  wires:
  previous/1 -> [previous_step]
  [previous_step] -> Step error/2
  [previous_step] -> Apply step/2
  target/1 -> Limit setpoint/1(u)
  limit/1 -> Limit setpoint/2(maximum)
  Limit setpoint/1(limited) -> Step error/1
  Step error/1 -> Limit rate/1(u)
  rate/1 -> Step time/1
  Step time/1 -> Limit rate/2(maximum)
  Limit rate/1(limited) -> Apply step/1
  Apply step/1 -> reference/1

== system odrive_foc/FOC Motion Controller/FOC Current Loop/Clarke and Park/Park rotation ==
  stationary : Inport
  cos_sin : Inport  Port=2
  Component 1 : DotProduct  OutDataTypeStr=Inherit: Inherit via internal rule
  Component 2 : DotProduct  OutDataTypeStr=Inherit: Inherit via internal rule
  Rotate vector : Mux  Inputs=2
  Rotation row 1 : Gain  Gain=single(eye(2))  Multiplication=Matrix(K*u) (u vector)
  Rotation row 2 : Gain  Gain=single([0 -1; 1 0])  Multiplication=Matrix(K*u) (u vector)
  rotating : Outport
  wires:
  stationary/1 -> [components_in]
  [components_in] -> Component 1/1
  [components_in] -> Component 2/1
  cos_sin/1 -> Rotation row 1/1, Rotation row 2/1
  Rotation row 1/1 -> Component 1/2
  Rotation row 2/1 -> Component 2/2
  Component 1/1 -> Rotate vector/1
  Component 2/1 -> Rotate vector/2
  Rotate vector/1 -> rotating/1

== system odrive_foc/FOC Motion Controller/FOC Current Loop/Current PI/Clamp PI output ==
  u : Inport
  maximum : Inport  Port=2
  Clamp u : simulink/Discontinuities/Saturation Dynamic  OutMin=[]  OutMax=[]  OutDataTypeStr=Inherit: Same as second input  OutDataType=fixdt(1, 16)  OutScaling=2^-10  DoSatur=off
  Negative limit : Gain  Gain=single(-1)
  limited : Outport
  wires:
  maximum/1 -> Clamp u/1, Negative limit/1
  u/1 -> Clamp u/2
  Negative limit/1 -> Clamp u/3
  Clamp u/1 -> limited/1

== system odrive_foc/FOC Motion Controller/FOC Current Loop/Current PI/Clamp candidate ==
  u : Inport
  maximum : Inport  Port=2
  Clamp u : simulink/Discontinuities/Saturation Dynamic  OutMin=[]  OutMax=[]  OutDataTypeStr=Inherit: Same as second input  OutDataType=fixdt(1, 16)  OutScaling=2^-10  DoSatur=off
  Negative limit : Gain  Gain=single(-1)
  limited : Outport
  wires:
  maximum/1 -> Clamp u/1, Negative limit/1
  u/1 -> Clamp u/2
  Negative limit/1 -> Clamp u/3
  Clamp u/1 -> limited/1

== system odrive_foc/FOC Motion Controller/FOC Current Loop/Current PI/Conditional integration ==
  p : Inport
  i_candidate : Inport  Port=2
  i_previous : Inport  Port=3
  error : Inport  Port=4
  maximum : Inport  Port=5
  Allow integral update : Logic  Operator=OR
  Candidate output : Sum
  Error unwinds : RelationalOperator  Operator=<
  Magnitude : Abs
  Output times error : Product  Inputs=**
  Select integral : Switch  Criteria=u2 ~= 0
  Within limit : RelationalOperator  Operator=<=
  Zero : Constant  Value=single(0)
  i_next : Outport
  wires:
  p/1 -> Candidate output/1
  i_candidate/1 -> Candidate output/2, Select integral/1
  Candidate output/1 -> Magnitude/1, Output times error/1
  Magnitude/1 -> Within limit/1
  maximum/1 -> Within limit/2
  error/1 -> Output times error/2
  Output times error/1 -> Error unwinds/1
  Zero/1 -> Error unwinds/2
  Within limit/1 -> Allow integral update/1
  Error unwinds/1 -> Allow integral update/2
  Allow integral update/1 -> Select integral/2
  i_previous/1 -> Select integral/3
  Select integral/1 -> i_next/1

== system odrive_foc/FOC Motion Controller/FOC Current Loop/Inverse Park and SVPWM/Common mode ==
  phase_volts : Inport
  Average : Gain  Gain=single(0.5)
  Peak : MinMax  Function=max
  Peak plus valley : Sum
  Valley : MinMax
  common_voltage : Outport
  wires:
  phase_volts/1 -> Peak/1, Valley/1
  Peak/1 -> Peak plus valley/1
  Valley/1 -> Peak plus valley/2
  Peak plus valley/1 -> Average/1
  Average/1 -> common_voltage/1

== system odrive_foc/FOC Motion Controller/FOC Current Loop/Inverse Park and SVPWM/Inverse Park rotation ==
  rotating : Inport
  cos_sin : Inport  Port=2
  Component 1 : DotProduct  OutDataTypeStr=Inherit: Inherit via internal rule
  Component 2 : DotProduct  OutDataTypeStr=Inherit: Inherit via internal rule
  Rotate vector : Mux  Inputs=2
  Rotation row 1 : Gain  Gain=single([1 0; 0 -1])  Multiplication=Matrix(K*u) (u vector)
  Rotation row 2 : Gain  Gain=single([0 1; 1 0])  Multiplication=Matrix(K*u) (u vector)
  stationary : Outport
  wires:
  rotating/1 -> [components_in]
  [components_in] -> Component 1/1
  [components_in] -> Component 2/1
  cos_sin/1 -> Rotation row 1/1, Rotation row 2/1
  Rotation row 1/1 -> Component 1/2
  Rotation row 2/1 -> Component 2/2
  Component 1/1 -> Rotate vector/1
  Component 2/1 -> Rotate vector/2
  Rotate vector/1 -> stationary/1

== system odrive_foc/FOC Motion Controller/FOC Current Loop/Voltage vector limit/Clamp new integral ==
  u : Inport
  maximum : Inport  Port=2
  Clamp u : simulink/Discontinuities/Saturation Dynamic  OutMin=[]  OutMax=[]  OutDataTypeStr=Inherit: Same as second input  OutDataType=fixdt(1, 16)  OutScaling=2^-10  DoSatur=off
  Negative limit : Gain  Gain=single(-1)
  limited : Outport
  wires:
  maximum/1 -> Clamp u/1, Negative limit/1
  u/1 -> Clamp u/2
  Negative limit/1 -> Clamp u/3
  Clamp u/1 -> limited/1

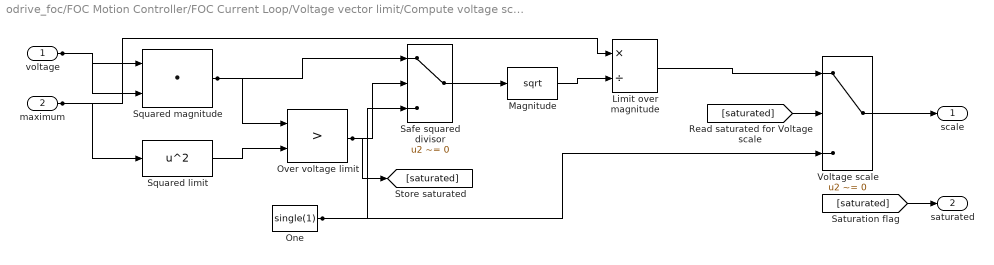
== system odrive_foc/FOC Motion Controller/FOC Current Loop/Voltage vector limit/Compute voltage scale ==
  voltage : Inport
  maximum : Inport  Port=2
  Limit over magnitude : Product  Inputs=*/
  Magnitude : Sqrt
  One : Constant  Value=single(1)
  Over voltage limit : RelationalOperator  Operator=>
  Safe squared divisor : Switch  Criteria=u2 ~= 0
  Squared limit : Math  Operator=square
  Squared magnitude : DotProduct  OutDataTypeStr=Inherit: Inherit via internal rule
  Voltage scale : Switch  Criteria=u2 ~= 0
  scale : Outport
  saturated : Outport  Port=2
  wires:
  Over voltage limit/1 -> [saturated], Safe squared divisor/2
  [saturated] -> Voltage scale/2
  [saturated] -> saturated/1
  voltage/1 -> Squared magnitude/1, Squared magnitude/2
  maximum/1 -> Squared limit/1, Limit over magnitude/1
  Squared magnitude/1 -> Over voltage limit/1, Safe squared divisor/1
  Squared limit/1 -> Over voltage limit/2
  One/1 -> Safe squared divisor/3, Voltage scale/3
  Safe squared divisor/1 -> Magnitude/1
  Magnitude/1 -> Limit over magnitude/2
  Limit over magnitude/1 -> Voltage scale/1
  Voltage scale/1 -> scale/1

== system odrive_foc/FOC Motion Controller/Motion loops/Speed PI/Clamp PI output ==
  u : Inport
  maximum : Inport  Port=2
  Clamp u : simulink/Discontinuities/Saturation Dynamic  OutMin=[]  OutMax=[]  OutDataTypeStr=Inherit: Same as second input  OutDataType=fixdt(1, 16)  OutScaling=2^-10  DoSatur=off
  Negative limit : Gain  Gain=single(-1)
  limited : Outport
  wires:
  maximum/1 -> Clamp u/1, Negative limit/1
  u/1 -> Clamp u/2
  Negative limit/1 -> Clamp u/3
  Clamp u/1 -> limited/1

== system odrive_foc/FOC Motion Controller/Motion loops/Speed PI/Clamp candidate ==
  u : Inport
  maximum : Inport  Port=2
  Clamp u : simulink/Discontinuities/Saturation Dynamic  OutMin=[]  OutMax=[]  OutDataTypeStr=Inherit: Same as second input  OutDataType=fixdt(1, 16)  OutScaling=2^-10  DoSatur=off
  Negative limit : Gain  Gain=single(-1)
  limited : Outport
  wires:
  maximum/1 -> Clamp u/1, Negative limit/1
  u/1 -> Clamp u/2
  Negative limit/1 -> Clamp u/3
  Clamp u/1 -> limited/1

== system odrive_foc/FOC Motion Controller/Motion loops/Speed PI/Conditional integration ==
  p : Inport
  i_candidate : Inport  Port=2
  i_previous : Inport  Port=3
  error : Inport  Port=4
  maximum : Inport  Port=5
  Allow integral update : Logic  Operator=OR
  Candidate output : Sum
  Error unwinds : RelationalOperator  Operator=<
  Magnitude : Abs
  Output times error : Product  Inputs=**
  Select integral : Switch  Criteria=u2 ~= 0
  Within limit : RelationalOperator  Operator=<=
  Zero : Constant  Value=single(0)
  i_next : Outport
  wires:
  p/1 -> Candidate output/1
  i_candidate/1 -> Candidate output/2, Select integral/1
  Candidate output/1 -> Magnitude/1, Output times error/1
  Magnitude/1 -> Within limit/1
  maximum/1 -> Within limit/2
  error/1 -> Output times error/2
  Output times error/1 -> Error unwinds/1
  Zero/1 -> Error unwinds/2
  Within limit/1 -> Allow integral update/1
  Error unwinds/1 -> Allow integral update/2
  Allow integral update/1 -> Select integral/2
  i_previous/1 -> Select integral/3
  Select integral/1 -> i_next/1

== system odrive_foc/FOC Motion Controller/Motion loops/Speed and acceleration limits/Limit rate ==
  u : Inport
  maximum : Inport  Port=2
  Clamp u : simulink/Discontinuities/Saturation Dynamic  OutMin=[]  OutMax=[]  OutDataTypeStr=Inherit: Same as second input  OutDataType=fixdt(1, 16)  OutScaling=2^-10  DoSatur=off
  Negative limit : Gain  Gain=single(-1)
  limited : Outport
  wires:
  maximum/1 -> Clamp u/1, Negative limit/1
  u/1 -> Clamp u/2
  Negative limit/1 -> Clamp u/3
  Clamp u/1 -> limited/1

== system odrive_foc/FOC Motion Controller/Motion loops/Speed and acceleration limits/Limit setpoint ==
  u : Inport
  maximum : Inport  Port=2
  Clamp u : simulink/Discontinuities/Saturation Dynamic  OutMin=[]  OutMax=[]  OutDataTypeStr=Inherit: Same as second input  OutDataType=fixdt(1, 16)  OutScaling=2^-10  DoSatur=off
  Negative limit : Gain  Gain=single(-1)
  limited : Outport
  wires:
  maximum/1 -> Clamp u/1, Negative limit/1
  u/1 -> Clamp u/2
  Negative limit/1 -> Clamp u/3
  Clamp u/1 -> limited/1

== system odrive_foc/FOC Motion Controller/Motion loops/Torque current and slew limits/Limit rate ==
  u : Inport
  maximum : Inport  Port=2
  Clamp u : simulink/Discontinuities/Saturation Dynamic  OutMin=[]  OutMax=[]  OutDataTypeStr=Inherit: Same as second input  OutDataType=fixdt(1, 16)  OutScaling=2^-10  DoSatur=off
  Negative limit : Gain  Gain=single(-1)
  limited : Outport
  wires:
  maximum/1 -> Clamp u/1, Negative limit/1
  u/1 -> Clamp u/2
  Negative limit/1 -> Clamp u/3
  Clamp u/1 -> limited/1

== system odrive_foc/FOC Motion Controller/Motion loops/Torque current and slew limits/Limit setpoint ==
  u : Inport
  maximum : Inport  Port=2
  Clamp u : simulink/Discontinuities/Saturation Dynamic  OutMin=[]  OutMax=[]  OutDataTypeStr=Inherit: Same as second input  OutDataType=fixdt(1, 16)  OutScaling=2^-10  DoSatur=off
  Negative limit : Gain  Gain=single(-1)
  limited : Outport
  wires:
  maximum/1 -> Clamp u/1, Negative limit/1
  u/1 -> Clamp u/2
  Negative limit/1 -> Clamp u/3
  Clamp u/1 -> limited/1
